simulink model "sf_change_model"  (R2025b)
settings: Solver=VariableStepAuto  StartTime=0.0  StopTime=inf  RelTol=1e-3
settings Model: Creator=The MathWorks, Inc.  LastModifiedBy=The MathWorks, Inc.
settings SolverCC: AlgebraicLoopSolver=TrustRegion
settings DataIOCC: ReturnWorkspaceOutputs=off
settings OptimizationCC: ReuseModelBlockBuffer=off
settings DebuggingCC: UnconnectedInputMsg=warning  UnconnectedOutputMsg=warning  UnconnectedLineMsg=warning  ArithmeticOperatorsInVariantConditions=warning
settings ModelReferenceCC: EnableRefExpFcnMdlSchedulingChecks=on
settings SFSimCC: CustomCodeUndefinedFunction=UseInterfaceOnly
settings RTWCC: GPUComputeCapability=3.5

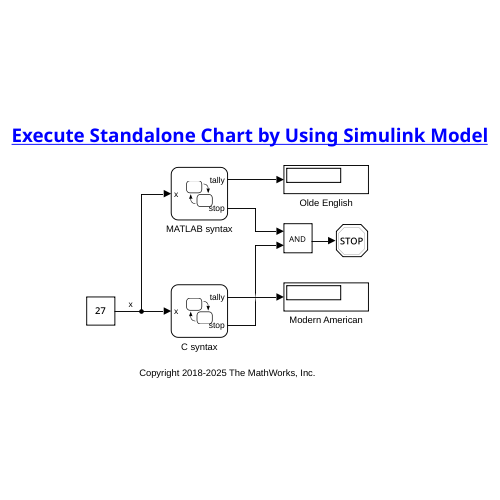
[thumbnail: Simulink's stored preview of the top-level diagram]
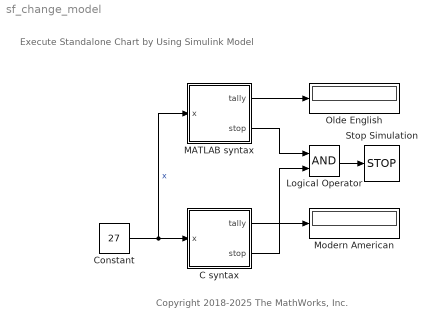
== system sf_change_model ==
  note: Copyright 2018-2025 The MathWorks, Inc.
  note: Execute Standalone Chart by Using Simulink Model
  C syntax : Stateflow chart  TreatAsAtomicUnit=on
  Constant : Constant  Value=27  OutDataTypeStr=int32
  Logical Operator : Logic  AllPortsSameDT=off  OutDataTypeStr=boolean
  MATLAB syntax : Stateflow chart  TreatAsAtomicUnit=on
  Modern American : Display
  Olde English : Display
  Stop Simulation : Stop
  wires:
  Constant/1 -> MATLAB syntax/1(x), C syntax/1(x)  "x"
  MATLAB syntax/1(tally) -> Olde English/1
  Logical Operator/1 -> Stop Simulation/1
  MATLAB syntax/2(stop) -> Logical Operator/1
  C syntax/2(stop) -> Logical Operator/2
  C syntax/1(tally) -> Modern American/1

== stateflow chart sf_change_model/C syntax ==
  state Initialize
    chartObj = ml('sf_change(''x'',%d,''coinValues'',[2 3 7],''coinNames'',{''Safety'' ''FieldGoal'' ''TouchDown''},''quietMode'',true,''-warningOnUninitializedData'',false)',x);
    tally = 0;
    done = false;
    stop = false;
  state Execute
    ml.step(chartObj);
    tally = ml.get(chartObj,'tally');
    done = ml.get(chartObj,'done');
  state Finish
    en:
    ml.disp(ml.get(chartObj,'tabula'));
    stop = true;
  (default) -> Initialize
  Initialize -> Execute
  Execute -> Finish : [done]
  data: x input int32; tally output double size=1; stop output; done local boolean size=1; chartObj local ml

== stateflow chart sf_change_model/MATLAB syntax ==
  state Initialize
    coder.extrinsic('sf_change');
    chartObj = sf_change('x',x,'coinValues',[1 12 24],'coinNames',{'Pennies' 'Shillings' 'Florins'},'quietMode',true,'-warningOnUninitializedData',false);
    tally = 0;
    done = false;
    stop = false;
  state Execute
    step(chartObj);
    tally = get(chartObj,'tally');
    done = get(chartObj,'done');
  state Finish
    en:
    disp(get(chartObj,'tabula'));
    stop = true;
  (default) -> Initialize
  Initialize -> Execute
  Execute -> Finish : [done]
  data: x input int32; tally output double size=1; chartObj local; stop output; done local boolean
